simulink model "tg9"  (R2022a)
settings: Solver=ode15s  StartTime=0.0  StopTime=10  MaxStep=0.01  RelTol=1e-3
InitFcn:
  | mecha_param2
  | control_param0
values from neighbouring files (symbols this model uses):
  b0 = 0    [sim_IMMC.m]
  b1 = 1    [sim_IMMC.m]
  back0 = 0    [sim_IMMC.m]
  back1 = 0    [sim_IMMC.m]
  boff = 0    [sim_IMMC.m]
  bon = 0    [sim_IMMC.m]
  c = 0.05    [mecha_param2.m]
  c_jointstop = 0.3 / (pi/180)    (= 17.1887338539)    [mecha_param2.m]
  calctalus = sqrt((L_foot - (DJ1x_foot))^2 + (H_foot-r_cs)^2)    [mecha_param2.m]
  calctoes = sqrt((H_foot-r_cs)^2 + (DJ1x_foot)^2)    [mecha_param2.m]
  corrD = 0.001    [control_param0.m]
  DG_HAT = 0.35    [mecha_param2.m]
  DG_thigh = 0.28    [mecha_param2.m]
  DJ1x_foot = 0.16-r_cs    (= 0.135)    [mecha_param2.m]
  eref = 0.04    [mecha_param2.m]
  FmaxBFSH = 350    [mecha_param2.m]
  FmaxGAS = 1500    [mecha_param2.m]
  FmaxGLU = 1500    [mecha_param2.m]
  FmaxHAM = 3000    [mecha_param2.m]
  FmaxHFL = 2000    [mecha_param2.m]
  FmaxRF = 1200    [mecha_param2.m]
  FmaxSOL = 4000    [mecha_param2.m]
  FmaxTA = 800    [mecha_param2.m]
  FmaxVAS = 6000    [mecha_param2.m]
  g = 9.81    [mecha_param2.m]
  g0 = 0    [sim_IMMC.m]
  g1 = 0    [sim_IMMC.m]
  H_foot = 0.08    [mecha_param2.m]
  In_HAT = 3    [mecha_param2.m]
  In_shank = 0.05    [mecha_param2.m]
  In_thigh = 0.15    [mecha_param2.m]
  K = 5    [mecha_param2.m]
  knee_thigh = [0 0 -(L_thigh/2)]    [mecha_param2.m]
  Kpress = m_HAT * g / DeltaThRef    (= 104967)    [mecha_param2.m]
  L_foot = 0.2    [mecha_param2.m]
  L_HAT = 0.8    [mecha_param2.m]
  L_shank = 0.46    [mecha_param2.m]
  L_thigh = 0.46    [mecha_param2.m]
  LoHAM = table2array(mt('LoHAM', 1))    [control_param0.m]
  LoHFL = table2array(mt('LoHFL', 1))    [control_param0.m]
  longD = longD - corrD    (= 0.019)    [control_param0.m]
  loptBFSH = 0.12    [mecha_param2.m]
  loptGAS = 0.05    [mecha_param2.m]
  loptGLU = 0.11    [mecha_param2.m]
  loptHAM = 0.10    (= 0.1)    [mecha_param2.m]
  loptHFL = 0.11    [mecha_param2.m]
  loptRF = 0.08    [mecha_param2.m]
  loptSOL = 0.04    [mecha_param2.m]
  loptTA = 0.06    [mecha_param2.m]
  loptVAS = 0.08    [mecha_param2.m]
  LoTA = table2array(mt('LoTA', 1))    [control_param0.m]
  lslackBFSH = 0.10    (= 0.1)    [mecha_param2.m]
  lslackGAS = 0.40    (= 0.4)    [mecha_param2.m]
  lslackGLU = 0.13    [mecha_param2.m]
  lslackHAM = 0.31    [mecha_param2.m]
  lslackHFL = 0.10    (= 0.1)    [mecha_param2.m]
  lslackRF = 0.35    [mecha_param2.m]
  lslackSOL = 0.26    [mecha_param2.m]
  lslackTA = 0.24    [mecha_param2.m]
  lslackVAS = 0.23    [mecha_param2.m]
  m_HAT = 53.5    [mecha_param2.m]
  m_shank = 3.5    [mecha_param2.m]
  m_thigh = 8.5    [mecha_param2.m]
  midD = midD - corrD    (= 0.009)    [control_param0.m]
  N = 1.5    [mecha_param2.m]
  nonoff = 0    [control_param0.m]
  phi_a_low = (70) * (pi / 180)    (= 1.2217304764)    [mecha_param2.m]
  phi_a_up = (130) * (pi / 180)    (= 2.26892802759)    [mecha_param2.m]
  phi_dl = 180    [mecha_param2.m]
  phi_h = 230 * (pi / 180)    (= 4.01425727959)    [mecha_param2.m]
  phi_k = 175 * (pi / 180)    (= 3.05432619099)    [mecha_param2.m]
  phictoes = asind((DJ1y_foot-r_cs)/calctoes)    [mecha_param2.m]
  phimaxGASa = 100*pi/180    (= 1.74532925199)    [mecha_param2.m]
  phimaxGASk = 140*pi/180    (= 2.44346095279)    [mecha_param2.m]
  phimaxRFk = 165*pi/180    (= 2.87979326579)    [mecha_param2.m]
  phimaxSOL = 100*pi/180    (= 1.74532925199)    [mecha_param2.m]
  phimaxTA = 80*pi/180    (= 1.3962634016)    [mecha_param2.m]
  phimaxVAS = 165*pi/180    (= 2.87979326579)    [mecha_param2.m]
  phirefBFSH = 160*pi/180    (= 2.79252680319)    [mecha_param2.m]
  phirefGASa = 80*pi/180    (= 1.3962634016)    [mecha_param2.m]
  phirefGASk = 165*pi/180    (= 2.87979326579)    [mecha_param2.m]
  phirefGLU = 120*pi/180    (= 2.09439510239)    [mecha_param2.m]
  phirefHAMh = 150*pi/180    (= 2.61799387799)    [mecha_param2.m]
  phirefHAMk = 180*pi/180    (= 3.14159265359)    [mecha_param2.m]
  phirefHFL = 160*pi/180    (= 2.79252680319)    [mecha_param2.m]
  phirefRFh = 170*pi/180    (= 2.96705972839)    [mecha_param2.m]
  phirefRFk = 125*pi/180    (= 2.18166156499)    [mecha_param2.m]
  phirefSOL = 90*pi/180    (= 1.57079632679)    [mecha_param2.m]
  phirefTA = 110*pi/180    (= 1.91986217719)    [mecha_param2.m]
  phirefVAS = 120*pi/180    (= 2.09439510239)    [mecha_param2.m]
  phiScaleGASa = acos(rGASamin/rGASamax)/(phiminGASa-phimaxGASa)    [mecha_param2.m]
  phiScaleGASk = acos(rGASkmin/rGASkmax)/(phiminGASk-phimaxGASk)    [mecha_param2.m]
  phiScaleRFk = acos(rRFkmin/rRFkmax)/(phiminRFk-phimaxRFk)    [mecha_param2.m]
  phiScaleSOL = acos(rSOLmin/rSOLmax)/(phiminSOL-phimaxSOL)    [mecha_param2.m]
  phiScaleTA = acos(rTAmin/rTAmax)/(phiminTA-phimaxTA)    [mecha_param2.m]
  phiScaleVAS = acos(rVASmin/rVASmax)/(phiminVAS-phimaxVAS)    [mecha_param2.m]
  r1 = 0    [sim_IMMC.m]
  r_cs = 0.025    [mecha_param2.m]
  rBFSH = 0.04    [mecha_param2.m]
  rGASamax = 0.06    [mecha_param2.m]
  rGASkmax = 0.05    [mecha_param2.m]
  rGLU = 0.08    [mecha_param2.m]
  rHAMh = 0.08    [mecha_param2.m]
  rHAMk = 0.05    [mecha_param2.m]
  rHFL = 0.08    [mecha_param2.m]
  rhoBFSH = 0.7    [mecha_param2.m]
  rhoGASa = 0.7    [mecha_param2.m]
  rhoGASk = 0.7    [mecha_param2.m]
  rhoGLU = 0.5    [mecha_param2.m]
  rhoHAMh = 0.5    [mecha_param2.m]
  rhoHAMk = 0.5    [mecha_param2.m]
  rhoHFL = 0.5    [mecha_param2.m]
  rhoRFh = 0.3    [mecha_param2.m]
  rhoRFk = 0.5    [mecha_param2.m]
  rhoSOL = 0.5    [mecha_param2.m]
  rhoTA = 0.7    [mecha_param2.m]
  rhoVAS = 0.6    [mecha_param2.m]
  rRFh = 0.08    [mecha_param2.m]
  rRFkmax = 0.06    [mecha_param2.m]
  rSOLmax = 0.06    [mecha_param2.m]
  ... (+25 more)
undefined symbols (not defined in the file or in its folder): beta11, beta12, beta13, beta14, beta15, beta16, beta21, beta22, beta23, beta24, beta25, beta26, beta31, beta32, beta33, beta34, beta35, beta36, beta41, beta42, beta43, beta44, beta45, beta46, beta51, beta52, beta53, beta54, beta55, beta56, betab1, betab2, betab3, betab4, betab5, betab6, betap11, betap12, betap13, betap14, betap15, betap16, betap21, betap22, betap23, betap24, betap25, betap26, betap31, betap32, betap33, betap34, betap35, betap36, betap41, betap42, betap43, betap44, betap45, betap46 ... (+102)
libraries: sm_lib x89, simulink x72, nesl_utility x58, simulink_extras x18
(part 7 of 12)

== system tg9/Muscle Actuation Layer/L VAS ==
  note: Left Vastus Musculo-Tendon Unit
  note: lmtu
  note: lmtu
  note: lce
  note: lce
  note: lce
  note: lce/lopt
  note: lse/lslack
  note: lse=lmtu-lce
  note: lceo = lmtu-lslack
  note: outcome fse is a proportion of fmax, because of that, it must be multiplied by fmax in order to get Fse
  note: Fmtc = Fse
  note: Fmax
  note: stimulation
  note: activation
  note: vce
  note: lce is the integration of vce over time using lopt as initial condition
  note: v[vmax] becomes v when *vmax and vce when *lopt
  note: STIM to A
  note: fv
  STIM : Inport
  lmtu [m] : Inport  Port=2
  BE force-length relation : Subsystem
  CE force-length relation : Subsystem
  CE inverse force-velocity relation : Subsystem
  Constant : Constant  Value=lslackVAS
  ECC TransferFcn : simulink_extras/Additional Linear/Transfer Fcn (with initial outputs)  N=[1]  D="[tau  1]"  Y0=preA  U0=0
  Fv = (Fse+Fbe) / (A*Fce+Fpe) : Product  Inputs=*/
  Gain : Gain  Gain=vmaxVAS*loptVAS
  Gain1 : Gain  Gain=1/lslackVAS
  Gain2 : Gain  Gain=1/loptVAS
  Gain3 : Gain  Gain=FmaxVAS
  Integrator : Integrator  InitialConditionSource=external  ZeroCross=off
  PE force-length relation : Subsystem
  Product : Product
  SE force-length relation : Subsystem
  Sum : Sum  Inputs=|+-
  Sum1 : Sum  Inputs=|-+
  Sum2 : Sum  Inputs=+|+
  Sum3 : Sum  Inputs=+|+
  excentric branch1 : Fcn  Commented=on  Expr=u(2) * (u(1)>1)*(u(1)<=u(3))
  Fmtc : Outport
  Lce : Outport  Port=2
  Vce : Outport  Port=3
  lse : Outport  Port=4
  A : Outport  Port=5
  fce [Fmax] : Outport  Port=6
  "fse [Fmax}" : Outport  Port=7
  wires:
  lmtu [m]/1 -> Sum1/2, Sum/1
  Integrator/1 -> Sum/2, Gain2/1, Lce/1
  Constant/1 -> Sum1/1
  Sum1/1 -> Integrator/2
  Gain/1 -> Vce/1, Integrator/1
  Sum/1 -> lse/1, Gain1/1
  Gain2/1 -> PE force-length relation/1(lce [lopt]), BE force-length relation/1(lce [lopt]), CE force-length relation/1(lce [lopt])
  Gain1/1 -> SE force-length relation/1(lse [lslack])
  SE force-length relation/1(fse [Fmax]) -> "fse [Fmax}"/1, Gain3/1, Sum2/1
  CE force-length relation/1(fce [Fmax]) -> fce [Fmax]/1, Product/1
  Product/1 -> Sum3/2
  STIM/1 -> ECC TransferFcn/1
  ECC TransferFcn/1 -> A/1, Product/2
  Gain3/1 -> Fmtc/1
  Sum2/1 -> Fv = (Fse+Fbe) / (A*Fce+Fpe)/1
  Sum3/1 -> Fv = (Fse+Fbe) / (A*Fce+Fpe)/2
  Fv = (Fse+Fbe) / (A*Fce+Fpe)/1 -> CE inverse force-velocity relation/1(Fv[Fmax])
  BE force-length relation/1(fbe [Fmax]) -> Sum2/2
  PE force-length relation/1(fpe [Fmax]) -> Sum3/1
  CE inverse force-velocity relation/1(v[vmax]) -> Gain/1

== system tg9/Muscle Actuation Layer/L VAS Link1 ==
  note: Muscle Length and Moment Arm
  phi23 [rad] : Inport
  Constant : Constant  Value=lslackVAS+loptVAS
  Constant1 : Constant  Value=phimaxVAS
  Constant2 : Constant  Value=phirefVAS
  Demux : Demux  Outputs=2
  Gain1 : Gain  Gain=rVASmax
  Gain3 : Gain  Gain=phiScaleVAS
  Gain4 : Gain  Gain=rhoVAS/phiScaleVAS
  Gain5 : Gain  Gain=phiScaleVAS
  Mux : Mux  Inputs=2
  Sum1 : Sum  Inputs=-+
  Sum2 : Sum  Inputs=|+-
  Sum3 : Sum  Inputs=-+|
  Sum5 : Sum  Inputs=|+-
  length change term : Trigonometry
  offset correction term : Trigonometry
  variable lever term : Trigonometry  Operator=cos
  lmtu [m] : Outport
  lever [m] : Outport  Port=2
  wires:
  Constant/1 -> Sum5/1
  Sum5/1 -> lmtu [m]/1
  phi23 [rad]/1 -> Sum3/2
  Sum3/1 -> Gain3/1
  Constant1/1 -> Sum3/1, Sum2/2
  Sum2/1 -> Gain5/1
  Constant2/1 -> Sum2/1
  length change term/1 -> Sum1/2
  offset correction term/1 -> Sum1/1
  Sum1/1 -> Mux/1
  variable lever term/1 -> Mux/2
  Mux/1 -> Gain1/1
  Gain1/1 -> Demux/1
  Demux/2 -> lever [m]/1
  Demux/1 -> Gain4/1
  Gain3/1 -> variable lever term/1, length change term/1
  Gain5/1 -> offset correction term/1
  Gain4/1 -> Sum5/2

== system tg9/Muscle Actuation Layer/L VAS Link2 ==
  note: Muscle Length and Moment Arm
  phi23 [rad] : Inport
  Constant : Constant  Value=lslackVAS+loptVAS
  Constant1 : Constant  Value=phimaxVAS
  Constant2 : Constant  Value=phirefVAS
  Demux : Demux  Outputs=2
  Gain1 : Gain  Gain=rVASmax
  Gain3 : Gain  Gain=phiScaleVAS
  Gain4 : Gain  Gain=rhoVAS/phiScaleVAS
  Gain5 : Gain  Gain=phiScaleVAS
  Mux : Mux  Inputs=2
  Sum1 : Sum  Inputs=-+
  Sum2 : Sum  Inputs=|+-
  Sum3 : Sum  Inputs=-+|
  Sum5 : Sum  Inputs=|+-
  length change term : Trigonometry
  offset correction term : Trigonometry
  variable lever term : Trigonometry  Operator=cos
  lmtu [m] : Outport
  lever [m] : Outport  Port=2
  wires:
  Constant/1 -> Sum5/1
  Sum5/1 -> lmtu [m]/1
  phi23 [rad]/1 -> Sum3/2
  Sum3/1 -> Gain3/1
  Constant1/1 -> Sum3/1, Sum2/2
  Sum2/1 -> Gain5/1
  Constant2/1 -> Sum2/1
  length change term/1 -> Sum1/2
  offset correction term/1 -> Sum1/1
  Sum1/1 -> Mux/1
  variable lever term/1 -> Mux/2
  Mux/1 -> Gain1/1
  Gain1/1 -> Demux/1
  Demux/2 -> lever [m]/1
  Demux/1 -> Gain4/1
  Gain3/1 -> variable lever term/1, length change term/1
  Gain5/1 -> offset correction term/1
  Gain4/1 -> Sum5/2

== system tg9/Muscle Actuation Layer/R Ankle Joint Limit ==
  note: Right Ankle Soft Limit
  phi [rad] : Inport
  dphi [rad/s] : Inport  Port=2
  Gain : Gain  Gain=c_jointstop
  Gain1 : Gain  Gain=1/w_max_jointstop
  Gain2 : Gain  Gain=-1
  Gain3 : Gain  Gain=c_jointstop
  Interval Test : simulink/Logic and Bit Operations/Interval Test  IntervalClosedRight=on  uplimit=phi_a_up + 40*pi/180  IntervalClosedLeft=on  lowlimit=phi_a_low - 40*pi/180  OutDataTypeStr=boolean
  Logical Operator : Logic  Operator=NOT  AllPortsSameDT=off  OutDataTypeStr=boolean
  Mux : Mux  Inputs=2
  Mux1 : Mux  Inputs=2
  Overextension torque : MATLAB Function  TreatAsAtomicUnit=on
  Overflexion torque : MATLAB Function  TreatAsAtomicUnit=on
  Stop Simulation : Stop
  Sum : Sum  Inputs=|+-
  Sum1 : Sum  Inputs=|+-
  Sum2 : Sum  Inputs=+|+
  overextension angle : Constant  Value=phi_a_up
  overflexion angle : Constant  Value=phi_a_low
  M_stop [Nm] : Outport
  wires:
  phi [rad]/1 -> Sum/1, Interval Test/1, Sum1/1
  overextension angle/1 -> Sum/2
  dphi [rad/s]/1 -> Gain1/1
  Sum/1 -> Gain/1
  Gain1/1 -> Mux1/2, Gain2/1
  Gain/1 -> Mux/1
  Gain2/1 -> Mux/2
  Mux/1 -> Overextension torque/1(u)
  Interval Test/1 -> Logical Operator/1
  Logical Operator/1 -> Stop Simulation/1
  Gain3/1 -> Mux1/1
  Sum1/1 -> Gain3/1
  overflexion angle/1 -> Sum1/2
  Overflexion torque/1(y) -> Sum2/2
  Mux1/1 -> Overflexion torque/1(u)
  Overextension torque/1(y) -> Sum2/1
  Sum2/1 -> M_stop [Nm]/1

== system tg9/Muscle Actuation Layer/R BFSH ==
  note: fv
  note: STIM to A
  note: v[vmax] becomes v when *vmax and vce when *lopt
  note: lce is the integration of vce over time using lopt as initial condition
  note: vce
  note: activation
  note: stimulation
  note: Fmax
  note: Fmtc = Fse
  note: outcome fse is a proportion of fmax, because of that, it must be multiplied by fmax in order to get Fse
  note: lceo = lmtu-lslack
  note: lse=lmtu-lce
  note: lse/lslack
  note: lce/lopt
  note: lce
  note: lce
  note: lce
  note: lmtu
  note: lmtu
  note: Left Biceps femoris short-head Musculo-Tendon Unit
  STIM : Inport
  lmtu [m] : Inport  Port=2
  BE force-length relation : Subsystem
  CE force-length relation : Subsystem
  CE inverse force-velocity relation : Subsystem
  Constant : Constant  Value=lslackBFSH
  ECC TransferFcn : simulink_extras/Additional Linear/Transfer Fcn (with initial outputs)  N=[1]  D="[tau  1]"  Y0=preA  U0=0
  Fv = (Fse+Fbe) / (A*Fce+Fpe) : Product  Inputs=*/
  Gain : Gain  Gain=vmaxBFSH*loptBFSH
  Gain1 : Gain  Gain=1/lslackBFSH
  Gain2 : Gain  Gain=1/loptBFSH
  Gain3 : Gain  Gain=FmaxBFSH
  Integrator : Integrator  InitialConditionSource=external  ZeroCross=off
  PE force-length relation : Subsystem
  Product : Product
  SE force-length relation : Subsystem
  Sum : Sum  Inputs=|+-
  Sum1 : Sum  Inputs=|-+
  Sum2 : Sum  Inputs=+|+
  Sum3 : Sum  Inputs=+|+
  excentric branch1 : Fcn  Commented=on  Expr=u(2) * (u(1)>1)*(u(1)<=u(3))
  Fmtc : Outport
  Lce : Outport  Port=2
  Vce : Outport  Port=3
  lse : Outport  Port=4
  A : Outport  Port=5
  fce [Fmax] : Outport  Port=6
  "fse [Fmax}" : Outport  Port=7
  wires:
  CE inverse force-velocity relation/1(v[vmax]) -> Gain/1
  PE force-length relation/1(fpe [Fmax]) -> Sum3/1
  BE force-length relation/1(fbe [Fmax]) -> Sum2/2
  Fv = (Fse+Fbe) / (A*Fce+Fpe)/1 -> CE inverse force-velocity relation/1(Fv[Fmax])
  Sum3/1 -> Fv = (Fse+Fbe) / (A*Fce+Fpe)/2
  Sum2/1 -> Fv = (Fse+Fbe) / (A*Fce+Fpe)/1
  Gain3/1 -> Fmtc/1
  ECC TransferFcn/1 -> Product/2, A/1
  STIM/1 -> ECC TransferFcn/1
  Product/1 -> Sum3/2
  CE force-length relation/1(fce [Fmax]) -> Product/1, fce [Fmax]/1
  SE force-length relation/1(fse [Fmax]) -> Sum2/1, Gain3/1, "fse [Fmax}"/1
  Gain1/1 -> SE force-length relation/1(lse [lslack])
  Gain2/1 -> CE force-length relation/1(lce [lopt]), BE force-length relation/1(lce [lopt]), PE force-length relation/1(lce [lopt])
  Sum/1 -> Gain1/1, lse/1
  Gain/1 -> Integrator/1, Vce/1
  Sum1/1 -> Integrator/2
  Constant/1 -> Sum1/1
  Integrator/1 -> Lce/1, Gain2/1, Sum/2
  lmtu [m]/1 -> Sum/1, Sum1/2

== system tg9/Muscle Actuation Layer/R GAS ==
  note: Left Gastrocnemius Musculo-Tendon Unit
  note: lmtu
  note: lmtu
  note: lce
  note: lce
  note: lce
  note: lce/lopt
  note: lse/lslack
  note: lse=lmtu-lce
  note: lceo = lmtu-lslack
  note: outcome fse is a proportion of fmax, because of that, it must be multiplied by fmax in order to get Fse
  note: Fmtc = Fse
  note: Fmax
  note: stimulation
  note: activation
  note: vce
  note: lce is the integration of vce over time using lopt as initial condition
  note: v[vmax] becomes v when *vmax and vce when *lopt
  note: STIM to A
  note: fv
  STIM : Inport
  lmtu [m] : Inport  Port=2
  BE force-length relation : Subsystem
  CE force-length relation : Subsystem
  CE inverse force-velocity relation : Subsystem
  Constant : Constant  Value=lslackGAS
  ECC TransferFcn : simulink_extras/Additional Linear/Transfer Fcn (with initial outputs)  N=[1]  D="[tau  1]"  Y0=preA  U0=0
  Fv = (Fse+Fbe) / (A*Fce+Fpe) : Product  Inputs=*/
  Gain : Gain  Gain=vmaxGAS*loptGAS
  Gain1 : Gain  Gain=1/lslackGAS
  Gain2 : Gain  Gain=1/loptGAS
  Gain3 : Gain  Gain=FmaxGAS
  Integrator : Integrator  InitialConditionSource=external  ZeroCross=off
  PE force-length relation : Subsystem
  Product : Product
  SE force-length relation : Subsystem
  Sum : Sum  Inputs=|+-
  Sum1 : Sum  Inputs=|-+
  Sum2 : Sum  Inputs=+|+
  Sum3 : Sum  Inputs=+|+
  excentric branch1 : Fcn  Commented=on  Expr=u(2) * (u(1)>1)*(u(1)<=u(3))
  Fmtc : Outport
  Lce : Outport  Port=2
  Vce : Outport  Port=3
  lse : Outport  Port=4
  A : Outport  Port=5
  fce [Fmax] : Outport  Port=6
  fse [Fmax] : Outport  Port=7
  wires:
  lmtu [m]/1 -> Sum1/2, Sum/1
  Integrator/1 -> Sum/2, Gain2/1, Lce/1
  Constant/1 -> Sum1/1
  Sum1/1 -> Integrator/2
  Gain/1 -> Vce/1, Integrator/1
  Sum/1 -> lse/1, Gain1/1
  Gain2/1 -> PE force-length relation/1(lce [lopt]), BE force-length relation/1(lce [lopt]), CE force-length relation/1(lce [lopt])
  Gain1/1 -> SE force-length relation/1(lse [lslack])
  SE force-length relation/1(fse [Fmax]) -> fse [Fmax]/1, Gain3/1, Sum2/1
  CE force-length relation/1(fce [Fmax]) -> fce [Fmax]/1, Product/1
  Product/1 -> Sum3/2
  STIM/1 -> ECC TransferFcn/1
  ECC TransferFcn/1 -> A/1, Product/2
  Gain3/1 -> Fmtc/1
  Sum2/1 -> Fv = (Fse+Fbe) / (A*Fce+Fpe)/1
  Sum3/1 -> Fv = (Fse+Fbe) / (A*Fce+Fpe)/2
  Fv = (Fse+Fbe) / (A*Fce+Fpe)/1 -> CE inverse force-velocity relation/1(Fv[Fmax])
  BE force-length relation/1(fbe [Fmax]) -> Sum2/2
  PE force-length relation/1(fpe [Fmax]) -> Sum3/1
  CE inverse force-velocity relation/1(v[vmax]) -> Gain/1

== system tg9/Muscle Actuation Layer/R GLU ==
  note: Left Gluteus Musculo-Tendon Unit
  note: lmtu
  note: lmtu
  note: lce
  note: lce
  note: lce
  note: lce/lopt
  note: lse/lslack
  note: lse=lmtu-lce
  note: lceo = lmtu-lslack
  note: outcome fse is a proportion of fmax, because of that, it must be multiplied by fmax in order to get Fse
  note: Fmtc = Fse
  note: Fmax
  note: stimulation
  note: activation
  note: vce
  note: lce is the integration of vce over time using lopt as initial condition
  note: v[vmax] becomes v when *vmax and vce when *lopt
  note: STIM to A
  note: fv
  STIM : Inport
  lmtu [m] : Inport  Port=2
  BE force-length relation : Subsystem
  CE force-length relation : Subsystem
  CE inverse force-velocity relation : Subsystem
  Constant : Constant  Value=lslackGLU
  ECC TransferFcn : simulink_extras/Additional Linear/Transfer Fcn (with initial outputs)  N=[1]  D="[tau  1]"  Y0=preA  U0=0
  Fv = (Fse+Fbe) / (A*Fce+Fpe) : Product  Inputs=*/
  Gain : Gain  Gain=vmaxGLU*loptGLU
  Gain1 : Gain  Gain=1/lslackGLU
  Gain2 : Gain  Gain=1/loptGLU
  Gain3 : Gain  Gain=FmaxGLU
  Integrator : Integrator  InitialConditionSource=external  ZeroCross=off
  PE force-length relation : Subsystem
  Product : Product
  SE force-length relation : Subsystem
  Sum : Sum  Inputs=|+-
  Sum1 : Sum  Inputs=|-+
  Sum2 : Sum  Inputs=+|+
  Sum3 : Sum  Inputs=+|+
  excentric branch1 : Fcn  Commented=on  Expr=u(2) * (u(1)>1)*(u(1)<=u(3))
  Fmtc : Outport
  Lce : Outport  Port=2
  Vce : Outport  Port=3
  lse : Outport  Port=4
  A : Outport  Port=5
  fce [Fmax] : Outport  Port=6
  fse [Fmax] : Outport  Port=7
  wires:
  lmtu [m]/1 -> Sum1/2, Sum/1
  Integrator/1 -> Sum/2, Gain2/1, Lce/1
  Constant/1 -> Sum1/1
  Sum1/1 -> Integrator/2
  Gain/1 -> Vce/1, Integrator/1
  Sum/1 -> lse/1, Gain1/1
  Gain2/1 -> PE force-length relation/1(lce [lopt]), BE force-length relation/1(lce [lopt]), CE force-length relation/1(lce [lopt])
  Gain1/1 -> SE force-length relation/1(lse [lslack])
  SE force-length relation/1(fse [Fmax]) -> fse [Fmax]/1, Gain3/1, Sum2/1
  CE force-length relation/1(fce [Fmax]) -> fce [Fmax]/1, Product/1
  Product/1 -> Sum3/2
  STIM/1 -> ECC TransferFcn/1
  ECC TransferFcn/1 -> A/1, Product/2
  Gain3/1 -> Fmtc/1
  Sum2/1 -> Fv = (Fse+Fbe) / (A*Fce+Fpe)/1
  Sum3/1 -> Fv = (Fse+Fbe) / (A*Fce+Fpe)/2
  Fv = (Fse+Fbe) / (A*Fce+Fpe)/1 -> CE inverse force-velocity relation/1(Fv[Fmax])
  BE force-length relation/1(fbe [Fmax]) -> Sum2/2
  PE force-length relation/1(fpe [Fmax]) -> Sum3/1
  CE inverse force-velocity relation/1(v[vmax]) -> Gain/1

== system tg9/Muscle Actuation Layer/R HAM1 ==
  note: Left Hamstrings Musculo-Tendon Unit
  note: lmtu
  note: lmtu
  note: lce
  note: lce
  note: lce
  note: lce/lopt
  note: lse/lslack
  note: lse=lmtu-lce
  note: lceo = lmtu-lslack
  note: outcome fse is a proportion of fmax, because of that, it must be multiplied by fmax in order to get Fse
  note: Fmtc = Fse
  note: Fmax
  note: stimulation
  note: activation
  note: vce
  note: lce is the integration of vce over time using lopt as initial condition
  note: v[vmax] becomes v when *vmax and vce when *lopt
  note: STIM to A
  note: fv
  STIM : Inport
  lmtu [m] : Inport  Port=2
  BE force-length relation : Subsystem
  CE force-length relation : Subsystem
  CE inverse force-velocity relation : Subsystem
  Constant : Constant  Value=lslackHAM
  ECC TransferFcn : simulink_extras/Additional Linear/Transfer Fcn (with initial outputs)  N=[1]  D="[tau  1]"  Y0=preA  U0=0
  Fv = (Fse+Fbe) / (A*Fce+Fpe) : Product  Inputs=*/
  Gain : Gain  Gain=vmaxHAM*loptHAM
  Gain1 : Gain  Gain=1/lslackHAM
  Gain2 : Gain  Gain=1/loptHAM
  Gain3 : Gain  Gain=FmaxHAM
  Integrator : Integrator  InitialConditionSource=external  ZeroCross=off
  PE force-length relation : Subsystem
  Product : Product
  SE force-length relation : Subsystem
  Sum : Sum  Inputs=|+-
  Sum1 : Sum  Inputs=|-+
  Sum2 : Sum  Inputs=+|+
  Sum3 : Sum  Inputs=+|+
  excentric branch1 : Fcn  Commented=on  Expr=u(2) * (u(1)>1)*(u(1)<=u(3))
  Fmtc : Outport
  Lce : Outport  Port=2
  Vce : Outport  Port=3
  lse : Outport  Port=4
  A : Outport  Port=5
  fce [Fmax] : Outport  Port=6
  fse [Fmax] : Outport  Port=7
  wires:
  lmtu [m]/1 -> Sum1/2, Sum/1
  Integrator/1 -> Sum/2, Gain2/1, Lce/1
  Constant/1 -> Sum1/1
  Sum1/1 -> Integrator/2
  Gain/1 -> Vce/1, Integrator/1
  Sum/1 -> lse/1, Gain1/1
  Gain2/1 -> PE force-length relation/1(lce [lopt]), BE force-length relation/1(lce [lopt]), CE force-length relation/1(lce [lopt])
  Gain1/1 -> SE force-length relation/1(lse [lslack])
  SE force-length relation/1(fse [Fmax]) -> fse [Fmax]/1, Gain3/1, Sum2/1
  CE force-length relation/1(fce [Fmax]) -> fce [Fmax]/1, Product/1
  Product/1 -> Sum3/2
  STIM/1 -> ECC TransferFcn/1
  ECC TransferFcn/1 -> A/1, Product/2
  Gain3/1 -> Fmtc/1
  Sum2/1 -> Fv = (Fse+Fbe) / (A*Fce+Fpe)/1
  Sum3/1 -> Fv = (Fse+Fbe) / (A*Fce+Fpe)/2
  Fv = (Fse+Fbe) / (A*Fce+Fpe)/1 -> CE inverse force-velocity relation/1(Fv[Fmax])
  BE force-length relation/1(fbe [Fmax]) -> Sum2/2
  PE force-length relation/1(fpe [Fmax]) -> Sum3/1
  CE inverse force-velocity relation/1(v[vmax]) -> Gain/1

== system tg9/Muscle Actuation Layer/R HFL ==
  note: Left Hip Flexor Group Musculo-Tendon Unit
  note: lmtu
  note: lmtu
  note: lce
  note: lce
  note: lce
  note: lce/lopt
  note: lse/lslack
  note: lse=lmtu-lce
  note: lceo = lmtu-lslack
  note: outcome fse is a proportion of fmax, because of that, it must be multiplied by fmax in order to get Fse
  note: Fmtc = Fse
  note: Fmax
  note: stimulation
  note: activation
  note: vce
  note: lce is the integration of vce over time using lopt as initial condition
  note: v[vmax] becomes v when *vmax and vce when *lopt
  note: STIM to A
  note: fv
  STIM : Inport
  lmtu [m] : Inport  Port=2
  BE force-length relation : Subsystem
  CE force-length relation : Subsystem
  CE inverse force-velocity relation : Subsystem
  Constant : Constant  Value=lslackHFL
  ECC TransferFcn : simulink_extras/Additional Linear/Transfer Fcn (with initial outputs)  N=[1]  D="[tau  1]"  Y0=preA  U0=0
  Fv = (Fse+Fbe) / (A*Fce+Fpe) : Product  Inputs=*/
  Gain : Gain  Gain=vmaxHFL*loptHFL
  Gain1 : Gain  Gain=1/lslackHFL
  Gain2 : Gain  Gain=1/loptHFL
  Gain3 : Gain  Gain=FmaxHFL
  Gain4 : Gain
  HFL : Scope
  Integrator : Integrator  InitialConditionSource=external  ZeroCross=off
  PE force-length relation : Subsystem
  Product : Product
  SE force-length relation : Subsystem
  Sum : Sum  Inputs=|+-
  Sum1 : Sum  Inputs=|-+
  Sum2 : Sum  Inputs=+|+
  Sum3 : Sum  Inputs=+|+
  excentric branch1 : Fcn  Commented=on  Expr=u(2) * (u(1)>1)*(u(1)<=u(3))
  Fmtc [N] : Outport
  Lce [m] : Outport  Port=2
  Vce [m/s] : Outport  Port=3
  lse [m] : Outport  Port=4
  A : Outport  Port=5
  Fce [N] : Outport  Port=6
  fse [Fmax] : Outport  Port=7
  wires:
  lmtu [m]/1 -> Sum1/2, Sum/1
  Integrator/1 -> Sum/2, Gain2/1, Lce [m]/1
  Constant/1 -> Sum1/1
  Sum1/1 -> Integrator/2
  Gain/1 -> Vce [m/s]/1, Integrator/1
  Sum/1 -> lse [m]/1, Gain1/1
  Gain2/1 -> PE force-length relation/1(lce [lopt]), BE force-length relation/1(lce [lopt]), CE force-length relation/1(lce [lopt])
  Gain1/1 -> SE force-length relation/1(lse [lslack])
  SE force-length relation/1(fse [Fmax]) -> fse [Fmax]/1, Gain3/1, Sum2/1
  CE force-length relation/1(fce [Fmax]) -> Product/1, Gain4/1
  Product/1 -> Sum3/2
  STIM/1 -> HFL/1, ECC TransferFcn/1
  ECC TransferFcn/1 -> A/1, Product/2
  Gain3/1 -> Fmtc [N]/1
  Sum2/1 -> Fv = (Fse+Fbe) / (A*Fce+Fpe)/1
  Sum3/1 -> Fv = (Fse+Fbe) / (A*Fce+Fpe)/2
  Fv = (Fse+Fbe) / (A*Fce+Fpe)/1 -> CE inverse force-velocity relation/1(Fv[Fmax])
  BE force-length relation/1(fbe [Fmax]) -> Sum2/2
  PE force-length relation/1(fpe [Fmax]) -> Sum3/1
  CE inverse force-velocity relation/1(v[vmax]) -> Gain/1
  Gain4/1 -> Fce [N]/1

== system tg9/Muscle Actuation Layer/R Hip Joint Limits ==
  note: Right Hip Soft Limit
  phi [rad] : Inport
  dphi [rad/s] : Inport  Port=2
  Gain : Gain  Gain=c_jointstop
  Gain1 : Gain  Gain=1/w_max_jointstop
  Gain2 : Gain  Gain=-1
  Interval Test : simulink/Logic and Bit Operations/Interval Test  IntervalClosedRight=on  uplimit=phi_h + 30*pi/180  IntervalClosedLeft=on  lowlimit=10*pi/180  OutDataTypeStr=boolean
  Logical Operator : Logic  Operator=NOT  AllPortsSameDT=off  OutDataTypeStr=boolean
  Mux : Mux  Inputs=2
  Overextension torque : MATLAB Function  TreatAsAtomicUnit=on
  Stop Simulation : Stop
  Sum : Sum  Inputs=|+-
  overextension angle : Constant  Value=phi_h
  M_stop [Nm] : Outport
  wires:
  phi [rad]/1 -> Interval Test/1, Sum/1
  overextension angle/1 -> Sum/2
  dphi [rad/s]/1 -> Gain1/1
  Sum/1 -> Gain/1
  Gain1/1 -> Gain2/1
  Gain/1 -> Mux/1
  Gain2/1 -> Mux/2
  Mux/1 -> Overextension torque/1(u)
  Overextension torque/1(y) -> M_stop [Nm]/1
  Interval Test/1 -> Logical Operator/1
  Logical Operator/1 -> Stop Simulation/1

== system tg9/Muscle Actuation Layer/R Knee Joint Limits ==
  note: Right Knee Soft Limit
  phi [rad] : Inport
  dphi [rad/s] : Inport  Port=2
  Gain : Gain  Gain=c_jointstop
  Gain1 : Gain  Gain=1/w_max_jointstop
  Gain2 : Gain  Gain=-1
  Interval Test : simulink/Logic and Bit Operations/Interval Test  IntervalClosedRight=on  uplimit=185*pi/180  IntervalClosedLeft=on  lowlimit=40*pi/180  OutDataTypeStr=boolean
  Logical Operator : Logic  Operator=NOT  AllPortsSameDT=off  OutDataTypeStr=boolean
  Mux : Mux  Inputs=2
  Overextension torque : MATLAB Function  TreatAsAtomicUnit=on
  Stop Simulation : Stop
  Sum : Sum  Inputs=|+-
  overextension angle : Constant  Value=phi_k
  M_stop [Nm] : Outport
  tag scope: KneeR_pain=global
  wires:
  phi [rad]/1 -> Interval Test/1, Sum/1
  overextension angle/1 -> Sum/2
  dphi [rad/s]/1 -> Gain1/1
  Sum/1 -> Gain/1
  Gain1/1 -> Gain2/1
  Gain/1 -> Mux/1
  Gain2/1 -> Mux/2
  Mux/1 -> Overextension torque/1(u)
  Overextension torque/1(y) -> [KneeR_pain], M_stop [Nm]/1
  Interval Test/1 -> Logical Operator/1
  Logical Operator/1 -> Stop Simulation/1

== system tg9/Muscle Actuation Layer/R RF ==
  note: fv
  note: STIM to A
  note: v[vmax] becomes v when *vmax and vce when *lopt
  note: lce is the integration of vce over time using lopt as initial condition
  note: vce
  note: activation
  note: stimulation
  note: Fmax
  note: Fmtc = Fse
  note: outcome fse is a proportion of fmax, because of that, it must be multiplied by fmax in order to get Fse
  note: lceo = lmtu-lslack
  note: lse=lmtu-lce
  note: lse/lslack
  note: lce/lopt
  note: lce
  note: lce
  note: lce
  note: lmtu
  note: lmtu
  note: Left Vastus Musculo-Tendon Unit
  STIM : Inport
  lmtu [m] : Inport  Port=2
  BE force-length relation : Subsystem
  CE force-length relation : Subsystem
  CE inverse force-velocity relation : Subsystem
  Constant : Constant  Value=lslackRF
  ECC TransferFcn : simulink_extras/Additional Linear/Transfer Fcn (with initial outputs)  N=[1]  D="[tau  1]"  Y0=preA  U0=0
  Fv = (Fse+Fbe) / (A*Fce+Fpe) : Product  Inputs=*/
  Gain : Gain  Gain=vmaxRF*loptRF
  Gain1 : Gain  Gain=1/lslackRF
  Gain2 : Gain  Gain=1/loptRF
  Gain3 : Gain  Gain=FmaxRF
  Integrator : Integrator  InitialConditionSource=external  ZeroCross=off
  PE force-length relation : Subsystem
  Product : Product
  SE force-length relation : Subsystem
  Sum : Sum  Inputs=|+-
  Sum1 : Sum  Inputs=|-+
  Sum2 : Sum  Inputs=+|+
  Sum3 : Sum  Inputs=+|+
  excentric branch1 : Fcn  Commented=on  Expr=u(2) * (u(1)>1)*(u(1)<=u(3))
  Fmtc : Outport
  Lce : Outport  Port=2
  Vce : Outport  Port=3
  lse : Outport  Port=4
  A : Outport  Port=5
  fce [Fmax] : Outport  Port=6
  "fse [Fmax}" : Outport  Port=7
  wires:
  CE inverse force-velocity relation/1(v[vmax]) -> Gain/1
  PE force-length relation/1(fpe [Fmax]) -> Sum3/1
  BE force-length relation/1(fbe [Fmax]) -> Sum2/2
  Fv = (Fse+Fbe) / (A*Fce+Fpe)/1 -> CE inverse force-velocity relation/1(Fv[Fmax])
  Sum3/1 -> Fv = (Fse+Fbe) / (A*Fce+Fpe)/2
  Sum2/1 -> Fv = (Fse+Fbe) / (A*Fce+Fpe)/1
  Gain3/1 -> Fmtc/1
  ECC TransferFcn/1 -> Product/2, A/1
  STIM/1 -> ECC TransferFcn/1
  Product/1 -> Sum3/2
  CE force-length relation/1(fce [Fmax]) -> Product/1, fce [Fmax]/1
  SE force-length relation/1(fse [Fmax]) -> Sum2/1, Gain3/1, "fse [Fmax}"/1
  Gain1/1 -> SE force-length relation/1(lse [lslack])
  Gain2/1 -> CE force-length relation/1(lce [lopt]), BE force-length relation/1(lce [lopt]), PE force-length relation/1(lce [lopt])
  Sum/1 -> Gain1/1, lse/1
  Gain/1 -> Integrator/1, Vce/1
  Sum1/1 -> Integrator/2
  Constant/1 -> Sum1/1
  Integrator/1 -> Lce/1, Gain2/1, Sum/2
  lmtu [m]/1 -> Sum/1, Sum1/2

== system tg9/Muscle Actuation Layer/R SOL ==
  note: Left Soleus Musculo-Tendon Unit
  note: lmtu
  note: lmtu
  note: lce
  note: lce
  note: lce
  note: lce/lopt
  note: lse/lslack
  note: lse=lmtu-lce
  note: lceo = lmtu-lslack
  note: outcome fse is a proportion of fmax, because of that, it must be multiplied by fmax in order to get Fse
  note: Fmtc = Fse
  note: Fmax
  note: stimulation
  note: activation
  note: vce
  note: lce is the integration of vce over time using lopt as initial condition
  note: v[vmax] becomes v when *vmax and vce when *lopt
  note: STIM to A
  note: fv
  STIM : Inport
  lmtu [m] : Inport  Port=2
  BE force-length relation : Subsystem
  CE force-length relation : Subsystem
  CE inverse force-velocity relation : Subsystem
  Constant : Constant  Value=lslackSOL
  ECC TransferFcn : simulink_extras/Additional Linear/Transfer Fcn (with initial outputs)  N=[1]  D="[tau  1]"  Y0=preA  U0=0
  Fv = (Fse+Fbe) / (A*Fce+Fpe) : Product  Inputs=*/
  Gain : Gain  Gain=vmaxSOL*loptSOL
  Gain1 : Gain  Gain=1/lslackSOL
  Gain2 : Gain  Gain=1/loptSOL
  Gain3 : Gain  Gain=FmaxSOL
  Integrator : Integrator  InitialConditionSource=external  ZeroCross=off
  PE force-length relation : Subsystem
  Product : Product
  SE force-length relation : Subsystem
  Sum : Sum  Inputs=|+-
  Sum1 : Sum  Inputs=|-+
  Sum2 : Sum  Inputs=+|+
  Sum3 : Sum  Inputs=+|+
  excentric branch1 : Fcn  Commented=on  Expr=u(2) * (u(1)>1)*(u(1)<=u(3))
  Fmtc : Outport
  Lce : Outport  Port=2
  Vce : Outport  Port=3
  lse : Outport  Port=4
  A : Outport  Port=5
  "fce [Fmax}" : Outport  Port=6
  "fse [Fmax}" : Outport  Port=7
  wires:
  lmtu [m]/1 -> Sum1/2, Sum/1
  Integrator/1 -> Sum/2, Gain2/1, Lce/1
  Constant/1 -> Sum1/1
  Sum1/1 -> Integrator/2
  Gain/1 -> Vce/1, Integrator/1
  Sum/1 -> lse/1, Gain1/1
  Gain2/1 -> PE force-length relation/1(lce [lopt]), BE force-length relation/1(lce [lopt]), CE force-length relation/1(lce [lopt])
  Gain1/1 -> SE force-length relation/1(lse [lslack])
  SE force-length relation/1(fse [Fmax]) -> "fse [Fmax}"/1, Gain3/1, Sum2/1
  CE force-length relation/1(fce [Fmax]) -> "fce [Fmax}"/1, Product/1
  Product/1 -> Sum3/2
  STIM/1 -> ECC TransferFcn/1
  ECC TransferFcn/1 -> A/1, Product/2
  Gain3/1 -> Fmtc/1
  Sum2/1 -> Fv = (Fse+Fbe) / (A*Fce+Fpe)/1
  Sum3/1 -> Fv = (Fse+Fbe) / (A*Fce+Fpe)/2
  Fv = (Fse+Fbe) / (A*Fce+Fpe)/1 -> CE inverse force-velocity relation/1(Fv[Fmax])
  BE force-length relation/1(fbe [Fmax]) -> Sum2/2
  PE force-length relation/1(fpe [Fmax]) -> Sum3/1
  CE inverse force-velocity relation/1(v[vmax]) -> Gain/1

== system tg9/Muscle Actuation Layer/R TA ==
  note: Left Tibialis Anterior Musculo-Tendon Unit
  note: lmtu
  note: lmtu
  note: lce
  note: lce
  note: lce
  note: lce/lopt
  note: lse/lslack
  note: lse=lmtu-lce
  note: lceo = lmtu-lslack
  note: outcome fse is a proportion of fmax, because of that, it must be multiplied by fmax in order to get Fse
  note: Fmtc = Fse
  note: Fmax
  note: stimulation
  note: activation
  note: vce
  note: lce is the integration of vce over time using lopt as initial condition
  note: v[vmax] becomes v when *vmax and vce when *lopt
  note: STIM to A
  note: fv
  STIM : Inport
  lmtu [m] : Inport  Port=2
  BE force-length relation : Subsystem
  CE force-length relation : Subsystem
  CE inverse force-velocity relation : Subsystem
  Constant : Constant  Value=lslackTA
  ECC TransferFcn : simulink_extras/Additional Linear/Transfer Fcn (with initial outputs)  N=[1]  D="[tau  1]"  Y0=preA  U0=0
  Fv = (Fse+Fbe) / (A*Fce+Fpe) : Product  Inputs=*/
  Gain : Gain  Gain=vmaxTA*loptTA
  Gain1 : Gain  Gain=1/lslackTA
  Gain2 : Gain  Gain=1/loptTA
  Gain3 : Gain  Gain=FmaxTA
  Integrator : Integrator  InitialConditionSource=external  ZeroCross=off
  PE force-length relation : Subsystem
  Product : Product
  SE force-length relation : Subsystem
  Sum : Sum  Inputs=|+-
  Sum1 : Sum  Inputs=|-+
  Sum2 : Sum  Inputs=+|+
  Sum3 : Sum  Inputs=+|+
  excentric branch1 : Fcn  Commented=on  Expr=u(2) * (u(1)>1)*(u(1)<=u(3))
  Fmtc : Outport
  Lce : Outport  Port=2
  Vce : Outport  Port=3
  lse : Outport  Port=4
  A : Outport  Port=5
  fce [Fmax] : Outport  Port=6
  fse [Fmax] : Outport  Port=7
  wires:
  lmtu [m]/1 -> Sum1/2, Sum/1
  Integrator/1 -> Sum/2, Gain2/1, Lce/1
  Constant/1 -> Sum1/1
  Sum1/1 -> Integrator/2
  Gain/1 -> Vce/1, Integrator/1
  Sum/1 -> lse/1, Gain1/1
  Gain2/1 -> PE force-length relation/1(lce [lopt]), BE force-length relation/1(lce [lopt]), CE force-length relation/1(lce [lopt])
  Gain1/1 -> SE force-length relation/1(lse [lslack])
  SE force-length relation/1(fse [Fmax]) -> fse [Fmax]/1, Gain3/1, Sum2/1
  CE force-length relation/1(fce [Fmax]) -> fce [Fmax]/1, Product/1
  Product/1 -> Sum3/2
  STIM/1 -> ECC TransferFcn/1
  ECC TransferFcn/1 -> A/1, Product/2
  Gain3/1 -> Fmtc/1
  Sum2/1 -> Fv = (Fse+Fbe) / (A*Fce+Fpe)/1
  Sum3/1 -> Fv = (Fse+Fbe) / (A*Fce+Fpe)/2
  Fv = (Fse+Fbe) / (A*Fce+Fpe)/1 -> CE inverse force-velocity relation/1(Fv[Fmax])
  BE force-length relation/1(fbe [Fmax]) -> Sum2/2
  PE force-length relation/1(fpe [Fmax]) -> Sum3/1
  CE inverse force-velocity relation/1(v[vmax]) -> Gain/1

== system tg9/Muscle Actuation Layer/R VAS ==
  note: Right Vastus Musculo-Tendon Unit
  note: lmtu
  note: lmtu
  note: lce
  note: lce
  note: lce
  note: lce/lopt
  note: lse/lslack
  note: lse=lmtu-lce
  note: lceo = lmtu-lslack
  note: outcome fse is a proportion of fmax, because of that, it must be multiplied by fmax in order to get Fse
  note: Fmtc = Fse
  note: Fmax
  note: stimulation
  note: activation
  note: vce
  note: lce is the integration of vce over time using lopt as initial condition
  note: v[vmax] becomes v when *vmax and vce when *lopt
  note: STIM to A
  note: fv
  STIM : Inport
  lmtu [m] : Inport  Port=2
  BE force-length relation : Subsystem
  CE force-length relation : Subsystem
  CE inverse force-velocity relation : Subsystem
  Constant : Constant  Value=lslackVAS
  ECC TransferFcn : simulink_extras/Additional Linear/Transfer Fcn (with initial outputs)  N=[1]  D="[tau  1]"  Y0=preA  U0=0
  Fv = (Fse+Fbe) / (A*Fce+Fpe) : Product  Inputs=*/
  Gain : Gain  Gain=vmaxVAS*loptVAS
  Gain1 : Gain  Gain=1/lslackVAS
  Gain2 : Gain  Gain=1/loptVAS
  Gain3 : Gain  Gain=FmaxVAS
  Integrator : Integrator  InitialConditionSource=external  ZeroCross=off
  PE force-length relation : Subsystem
  Product : Product
  SE force-length relation : Subsystem
  Sum : Sum  Inputs=|+-
  Sum1 : Sum  Inputs=|-+
  Sum2 : Sum  Inputs=+|+
  Sum3 : Sum  Inputs=+|+
  excentric branch1 : Fcn  Commented=on  Expr=u(2) * (u(1)>1)*(u(1)<=u(3))
  vasinput : Scope
  Fmtc : Outport
  Lce : Outport  Port=2
  Vce : Outport  Port=3
  lse : Outport  Port=4
  A : Outport  Port=5
  fce [Fmax] : Outport  Port=6
  fse [Fmax] : Outport  Port=7
  wires:
  lmtu [m]/1 -> Sum1/2, Sum/1
  Integrator/1 -> Sum/2, Gain2/1, Lce/1
  Constant/1 -> Sum1/1
  Sum1/1 -> Integrator/2
  Gain/1 -> Vce/1, Integrator/1
  Sum/1 -> lse/1, Gain1/1
  Gain2/1 -> PE force-length relation/1(lce [lopt]), BE force-length relation/1(lce [lopt]), CE force-length relation/1(lce [lopt])
  Gain1/1 -> SE force-length relation/1(lse [lslack])
  SE force-length relation/1(fse [Fmax]) -> fse [Fmax]/1, Gain3/1, Sum2/1
  CE force-length relation/1(fce [Fmax]) -> fce [Fmax]/1, Product/1
  Product/1 -> Sum3/2
  STIM/1 -> ECC TransferFcn/1
  ECC TransferFcn/1 -> A/1, Product/2
  Gain3/1 -> vasinput/1, Fmtc/1
  Sum2/1 -> Fv = (Fse+Fbe) / (A*Fce+Fpe)/1
  Sum3/1 -> Fv = (Fse+Fbe) / (A*Fce+Fpe)/2
  Fv = (Fse+Fbe) / (A*Fce+Fpe)/1 -> CE inverse force-velocity relation/1(Fv[Fmax])
  BE force-length relation/1(fbe [Fmax]) -> Sum2/2
  PE force-length relation/1(fpe [Fmax]) -> Sum3/1
  CE inverse force-velocity relation/1(v[vmax]) -> Gain/1

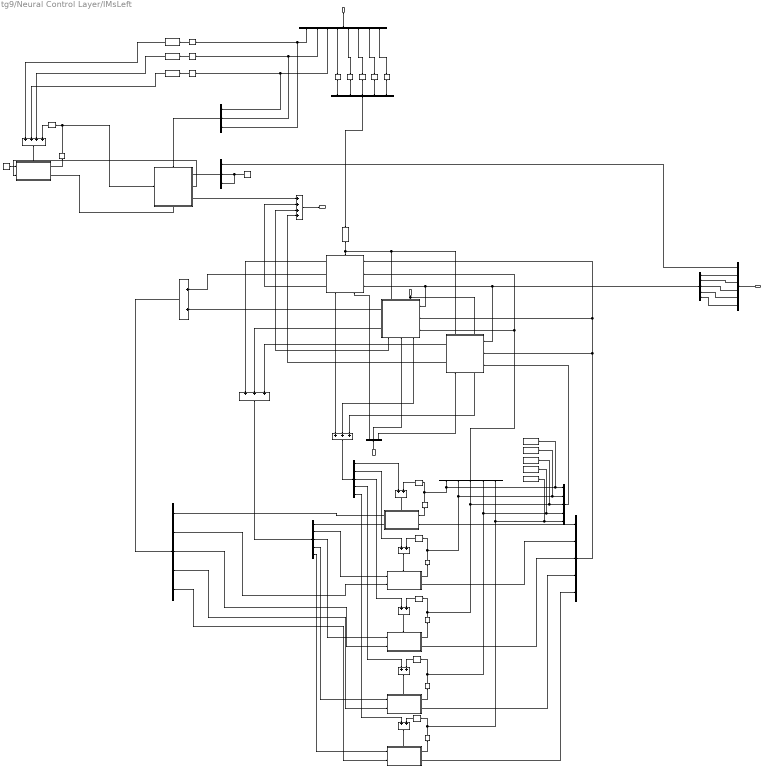
== system tg9/Neural Control Layer/IMsLeft ==
  triggers : Inport
  eta : Inport  Port=2
  drivers : Inport  Port=3
  right2left : Inport  Port=4
  Add{1..5,8} (6 alike) : Sum
  Add10 : Sum  Inputs=+++
  Add6 : Sum  Inputs=++++
  Add7 : Sum  Inputs=++++
  Add9 : Sum  Inputs=+++
  Bias{1..6} (6 alike) : Bias  Bias=-0.001  SaturateOnIntegerOverflow=off
  Cast To Double{,1..3} (4 alike) : DataTypeConversion  OutDataTypeStr=double  SaturateOnIntegerOverflow=off  RndMeth=Floor
  Demux : Demux  Outputs=6
  Demux1 : Demux  Outputs=5
  Demux2 : Demux  Outputs=5
  Demux3 : Demux  Outputs=3
  Demux4 : Demux  Outputs=5
  Demux5 : Demux  Outputs=8
  Hit Crossing{1..8} (8 alike) : HitCross  HitCrossingOffset=0.5  HitCrossingDirection=rising  ZeroCross=off
  IMx3 : Subsystem
      settings: PortSchema="{\"entries\":[{\"content\":{\"sides\":[{\"content\":{\"connectorIds\":[\"In1\"]},\"type\":\"ConnectorPlacement.EquallySpacedRectSide\",\"uuid\":\"605af916-6978-477d-a73f-0473cfddaa9b\"},{\"content\":{\"connectorIds\":[\"In4\",\"Out1\",\"Out2\"],\"side\":\"RIGHT\"},\"type\":\"ConnectorPlacement.EquallySpacedRectSide\",\"uuid\":\"ae4b258d-886c-42c2-bd45-f153a9ad36f8\"},{\"content\":{\"connectorIds\":[\"In2\"],\"side\":\"TOP\"},\"type\":\"ConnectorPlacement.EquallySpacedRectSide\",\"uuid\":\"4a03238d-2b6a-43dc-934f-97c6bc5fc8f2\"},{\"content\":{\"connectorIds\":[\"In3\"],\"side\":\"BOTTOM\"},\"type\":\"ConnectorPlacement.EquallySpacedRectSide\",\"uuid\":\"5d056236-5ce8-482a-98e4-2b75471ba733\"}]},\"type\":\"ConnectorPlacement.EquallySpacedConnector\",\"uuid\":\"c8afc41f-4e3a-4f48-b0c9-a380f8c80fc8\"}],\"packageUris\":[\"http://schema.mathworks.com/mf0/Connector/R2020b\"],\"version\":\"1.0\"}"
  Mux{,1..3,5} (5 alike) : Mux  Inputs=5
  Mux6 : Mux  Inputs=3
  Mux7 : Mux  Inputs=3
  S1 : Subsystem  TreatAsAtomicUnit=on
  S2 : Subsystem  TreatAsAtomicUnit=on
  S3 : Subsystem  TreatAsAtomicUnit=on
  S4 : Subsystem  TreatAsAtomicUnit=on
  S5 : Subsystem  TreatAsAtomicUnit=on
  Sx : Subsystem  TreatAsAtomicUnit=on
  To Workspace2 : ToWorkspace  VariableName=sync1  SampleTime=-1
  To Workspace3 : ToWorkspace  VariableName=sync2  SampleTime=-1
  To Workspace4 : ToWorkspace  VariableName=sync3  SampleTime=-1
  To Workspace5 : ToWorkspace  VariableName=sync4  SampleTime=-1
  To Workspace6 : ToWorkspace  VariableName=sync5  SampleTime=-1
  Transport Delay{1..6} (6 alike) : TransportDelay  DelayTime=corrD
  Zero : Constant  Value=0  OutDataTypeStr=Inherit: Inherit via back propagation
  backwardpool : Subsystem
      settings: PortSchema="{\"entries\":[{\"content\":{\"sides\":[{\"content\":{\"connectorIds\":[\"In1\",\"In2\",\"In3\"]},\"type\":\"ConnectorPlacement.EquallySpacedRectSide\",\"uuid\":\"a61b6c6e-9e6f-45f2-b50f-9bcdc7a13346\"},{\"content\":{\"connectorIds\":[\"Out1\",\"Out2\"],\"side\":\"RIGHT\"},\"type\":\"ConnectorPlacement.EquallySpacedRectSide\",\"uuid\":\"1e8eaab5-7abe-40b4-aee2-b3f1e694b70c\"},{\"content\":{\"connectorIds\":[\"In4\",\"In5\"],\"side\":\"TOP\"},\"type\":\"ConnectorPlacement.EquallySpacedRectSide\",\"uuid\":\"0d5c3f76-1ab4-4f7c-806d-755b82fcb7e0\"},{\"content\":{\"connectorIds\":[\"Out3\",\"In6\"],\"side\":\"BOTTOM\"},\"type\":\"ConnectorPlacement.EquallySpacedRectSide\",\"uuid\":\"6e4a109d-fd90-45a6-b737-e259d18310f6\"}]},\"type\":\"ConnectorPlacement.EquallySpacedConnector\",\"uuid\":\"c9455465-31f2-4bd0-89ee-d0d51ed162fd\"}],\"packageUris\":[\"http://schema.mathworks.com/mf0/Connector/R2020b\"],\"version\":\"1.0\"}"
  etas2 : Constant  OutDataTypeStr=Inherit: Inherit via back propagation
  forwardpool : Subsystem
      settings: PortSchema="{\"entries\":[{\"content\":{\"sides\":[{\"content\":{\"connectorIds\":[\"In1\",\"In2\",\"In3\"]},\"type\":\"ConnectorPlacement.EquallySpacedRectSide\",\"uuid\":\"a61b6c6e-9e6f-45f2-b50f-9bcdc7a13346\"},{\"content\":{\"connectorIds\":[\"Out1\",\"Out2\"],\"side\":\"RIGHT\"},\"type\":\"ConnectorPlacement.EquallySpacedRectSide\",\"uuid\":\"1e8eaab5-7abe-40b4-aee2-b3f1e694b70c\"},{\"content\":{\"connectorIds\":[\"In4\",\"In5\"],\"side\":\"TOP\"},\"type\":\"ConnectorPlacement.EquallySpacedRectSide\",\"uuid\":\"0d5c3f76-1ab4-4f7c-806d-755b82fcb7e0\"},{\"content\":{\"connectorIds\":[\"Out3\",\"In6\",\"Out4\"],\"side\":\"BOTTOM\"},\"type\":\"ConnectorPlacement.EquallySpacedRectSide\",\"uuid\":\"6e4a109d-fd90-45a6-b737-e259d18310f6\"}]},\"type\":\"ConnectorPlacement.EquallySpacedConnector\",\"uuid\":\"c9455465-31f2-4bd0-89ee-d0d51ed162fd\"}],\"packageUris\":[\"http://schema.mathworks.com/mf0/Connector/R2020b\"],\"version\":\"1.0\"}"
  standingpool : Subsystem
      settings: PortSchema="{\"entries\":[{\"content\":{\"sides\":[{\"content\":{\"connectorIds\":[\"In1\",\"In2\",\"In3\"]},\"type\":\"ConnectorPlacement.EquallySpacedRectSide\",\"uuid\":\"b712be9c-ffb9-40b3-9573-f9951c2c9790\"},{\"content\":{\"connectorIds\":[\"Out1\",\"Out2\",\"Out3\"],\"side\":\"RIGHT\"},\"type\":\"ConnectorPlacement.EquallySpacedRectSide\",\"uuid\":\"8b219718-e783-4b0c-8b79-845ed528538f\"},{\"content\":{\"connectorIds\":[\"In4\"],\"side\":\"TOP\"},\"type\":\"ConnectorPlacement.EquallySpacedRectSide\",\"uuid\":\"e04791c1-32da-4b4e-9c5c-e19faa0d0170\"},{\"content\":{\"connectorIds\":[\"In5\",\"Out4\"],\"side\":\"BOTTOM\"},\"type\":\"ConnectorPlacement.EquallySpacedRectSide\",\"uuid\":\"996429ae-f4aa-4411-9589-2ace4ffd34b2\"}]},\"type\":\"ConnectorPlacement.EquallySpacedConnector\",\"uuid\":\"20796571-eb07-4761-9f65-93ae0d0a6d2c\"}],\"packageUris\":[\"http://schema.mathworks.com/mf0/Connector/R2020b\"],\"version\":\"1.0\"}"
  beta : Outport
  wires:
  Transport Delay2/1 -> Mux2/4, To Workspace5/1, Mux5/4, Bias2/1
  Transport Delay1/1 -> Mux2/3, To Workspace4/1, Mux5/3, Bias3/1
  Transport Delay6/1 -> Mux2/2, To Workspace3/1, Mux5/2, Bias4/1
  Cast To Double/1 -> forwardpool/5(triggers), backwardpool/5(triggers), standingpool/4(triggers)
  standingpool/4(trigger_out) -> Add10/1
  Demux4/5 -> Add5/1
  Demux4/4 -> Add4/1
  Demux4/3 -> Add2/1
  Demux4/2 -> Add1/1
  Demux4/1 -> Add3/1
  Add10/1 -> Demux4/1
  forwardpool/3(trigger_out) -> Add10/2
  Mux3/1 -> Cast To Double/1
  Hit Crossing2/1 -> Mux3/1
  Hit Crossing1/1 -> Mux3/2
  Hit Crossing3/1 -> Mux3/3
  Hit Crossing4/1 -> Mux3/4
  Hit Crossing5/1 -> Mux3/5
  Demux5/8 -> Hit Crossing5/1
  Demux5/7 -> Hit Crossing4/1
  Demux5/6 -> Hit Crossing3/1
  Add5/1 -> S5/Enable
  Add4/1 -> S4/Enable
  Add2/1 -> S3/Enable
  Add1/1 -> S2/Enable
  Bias5/1 -> Add3/2
  Bias4/1 -> Add1/2
  Bias3/1 -> Add2/2
  Bias1/1 -> Add5/2
  Demux3/1 -> standingpool/5(control)
  Demux3/2 -> forwardpool/6(control)
  standingpool/2(phi) -> Add8/1
  forwardpool/1(phi) -> Add8/2
  Bias2/1 -> Add4/2
  drivers/1 -> Demux3/1
  Demux2/5 -> S5/1(varthetau)
  Demux2/4 -> S4/1(varthetau)
  Demux2/3 -> S3/1(varthetau)
  Demux2/2 -> S2/1(varthetau)
  Add8/1 -> Demux1/1
  Add9/1 -> Demux2/1
  Demux2/1 -> S1/2(varthetau)
  forwardpool/2(vartheta) -> Add9/2
  standingpool/1(vartheta) -> Add9/1
  Mux2/1 -> standingpool/2(ui), forwardpool/3(ui)
  Demux5/4 -> Hit Crossing2/1
  S5/1(u3) -> Transport Delay3/1
  Demux1/5 -> S5/2(phi)
  S5/2(theta) -> Mux1/5
  S4/2(theta) -> Mux1/4
  Demux1/4 -> S4/2(phi)
  S4/1(u3) -> Transport Delay2/1
  S3/1(u3) -> Transport Delay1/1
  S2/1(u2) -> Transport Delay6/1
  S1/1(u1) -> Transport Delay5/1
  Demux1/3 -> S3/2(phi)
  Demux1/2 -> S2/2(phi)
  Demux1/1 -> S1/1(phi)
  S3/2(theta) -> Mux1/3
  S2/2(theta) -> Mux1/2
  S1/2(theta) -> Mux1/1
  Mux1/1 -> backwardpool/2(phase), standingpool/1(phase), forwardpool/2(phase)
  triggers/1 -> Demux5/1
  Demux5/5 -> Hit Crossing1/1
  Mux/1 -> backwardpool/1(eta), forwardpool/1(eta), standingpool/3(eta)
  right2left/1 -> backwardpool/4(right2left), forwardpool/4(right2left)
  Add3/1 -> S1/Enable
  Add6/1 -> Sx/Enable
  Sx/1(u1) -> Transport Delay4/1
  Bias6/1 -> Add6/4
  Transport Delay4/1 -> IMx3/1(ui), Bias6/1
  Demux5/3 -> Mux7/1, Hit Crossing6/1
  Hit Crossing6/1 -> Cast To Double1/1
  Cast To Double1/1 -> Add6/2
  IMx3/1(vartheta) -> Sx/2(varthetau)
  Zero/1 -> Sx/1(phi)
  Sx/2(theta) -> IMx3/3(phase)
  Demux/3 -> Mux/2
  Demux/4 -> Mux/3
  Demux/5 -> Mux/4
  Demux/2 -> Mux/1
  Demux/6 -> Mux/5
  eta/1 -> Demux/1
  Demux5/2 -> Hit Crossing7/1, Mux7/2
  Hit Crossing7/1 -> Cast To Double2/1
  Cast To Double2/1 -> Add6/3
  Demux5/1 -> Hit Crossing8/1, Mux7/3
  Hit Crossing8/1 -> Cast To Double3/1
  Demux/1 -> Mux6/1
  Demux3/3 -> backwardpool/6(control)
  backwardpool/3(trigger_out) -> Add10/3
  backwardpool/1(vartheta) -> Add9/3
  Transport Delay3/1 -> Mux2/5, To Workspace6/1, Mux5/5, Bias1/1
  Mux5/1 -> backwardpool/3(ui)
  Mux6/1 -> IMx3/4(eta)
  etas2/1 -> Mux6/3, Mux6/2
  Cast To Double3/1 -> Add6/1
  Mux7/1 -> IMx3/2(drivers)
  IMx3/2(beta) -> Add7/1
  Add7/1 -> beta/1
  standingpool/3(beta) -> Add7/2
  Transport Delay5/1 -> Mux2/1, To Workspace2/1, Mux5/1, Bias5/1
  forwardpool/4(beta) -> Add7/3
  backwardpool/2(beta) -> Add7/4
